simulink model "FullFMS_2026_02_25_V0_4_29_R2025b"  (R2025b)
settings: Solver=FixedStepAuto  StartTime=0.0  StopTime=inf  FixedStep=0.01  MaxStep=0.01  RelTol=1e-2
PreLoadFcn:
  | load("BUS_CONFIG.mat")
libraries: opcualib x8
(part 4 of 4)

== matlab function FullFMS_2026_02_25_V0_4_29_R2025b/MATLAB Function ==
  data: u1 input boolean; u2 input boolean; u3 input boolean; u4 input boolean; u5 input boolean; u6 input boolean; u7 input boolean; u8 input boolean; u9 input boolean; u10 input boolean; u11 input boolean; u12 input boolean; u13 input boolean; u14 input boolean; u15 input boolean; u16 input boolean; u17 input boolean; u18 input boolean; u19 input boolean; u20 input boolean; u21 input boolean; u22 input boolean; u23 input boolean; u24 input boolean; u25 input boolean; u26 input boolean; u27 input boolean; u28 input boolean; u29 input boolean; u30 input boolean; u31 input boolean; u32 input boolean; u33 input boolean; u34 input boolean; u35 input boolean; u36 input boolean; u37 input boolean; u38 input boolean; u39 input boolean; u40 input boolean; u41 input boolean; u42 input boolean; u43 input boolean; u44 input boolean; u45 input boolean; u46 input boolean; u47 input boolean; u48 input boolean; u49 input boolean; u50 input boolean; u51 input boolean; u52 input boolean; u53 input boolean; u54 input boolean; u55 input boolean; u56 input boolean; u57 input boolean; u58 input boolean; u59 input boolean; u60 input boolean; u61 input boolean; u62 input boolean; u63 input boolean; u64 input boolean; u65 input boolean; u66 input boolean; F_22_Led_On output boolean; F_22_Led_Off output boolean; F_22_Conveyor output boolean; F_24_Release_FB output boolean; F_25_Release_FB output boolean; F_26_Release_FB output boolean; F_27_Release_FB output boolean; F_28_Release_FB output boolean; F_29_Release_FB output boolean; C_24_CartDel output boolean; C_24_CRoute_Out output boolean; C_24_Request output boolean; C_24_CRoute_In output boolean; C_25_CartDel output boolean; C_25_CRoute_Out output boolean; C_25_Request output boolean; C_25_CRoute_In output boolean; C_26_CartDel output boolean; C_26_CRoute_Out output boolean; C_26_Request output boolean; C_26_CRoute_In output boolean; C_27_CartDel output boolean; C_27_CRoute_Out output boolean; C_27_Request output boolean; C_27_CRoute_In output boolean; C_28_CartDel output boolean; C_28_CRoute_Out output boolean; C_28_Request output boolean; C_28_CRoute_In output boolean; C_29_CartDel output boolean; C_29_CRoute_Out output boolean; C_29_Request output boolean; C_29_CRoute_In output boolean; O_20_On output boolean; O_20_Off output boolean; O_20_Controler_On output boolean; O_24_Cart_Stat output boolean; O_24_Cart_Next output boolean; O_24_Optic output boolean; O_24_Count output boolean; O_24_Pist_Bck output boolean; O_25_Cart_Stat output boolean; O_25_Cart_Next output boolean; O_25_Optic output boolean; O_25_Count output boolean; O_25_Pist_Bck output boolean; O_26_Cart_Stat output boolean; O_26_Cart_Next output boolean; O_26_Optic output boolean; O_26_Count output boolean; O_26_Pist_Bck output boolean; O_27_Cart_Stat output boolean; O_27_Cart_Next output boolean; O_27_Optic output boolean; O_27_Count output boolean; O_27_Pist_Bck output boolean; O_28_Cart_Stat output boolean; O_28_Cart_Next output boolean; O_28_Optic output boolean; O_28_Count output boolean; O_28_Pist_Bck output boolean; O_29_Cart_Stat output boolean; O_29_Cart_Next output boolean; O_29_Optic output boolean; O_29_Count output boolean; O_29_Pist_Bck output boolean
function [F_22_Led_On,F_22_Led_Off,F_22_Conveyor,F_24_Release_FB,F_25_Release_FB,F_26_Release_FB,F_27_Release_FB,F_28_Release_FB,F_29_Release_FB,...
 C_24_CartDel,C_24_CRoute_Out,C_24_Request,C_24_CRoute_In,C_25_CartDel,C_25_CRoute_Out,C_25_Request,C_25_CRoute_In,C_26_CartDel,C_26_CRoute_Out,C_26_Request,C_26_CRoute_In,C_27_CartDel,C_27_CRoute_Out,C_27_Request,C_27_CRoute_In,C_28_CartDel,C_28_CRoute_Out,C_28_Request,C_28_CRoute_In,C_29_CartDel,C_29_CRoute_Out,C_29_Request,C_29_CRoute_In,...
 O_20_On,O_20_Off,O_20_Controler_On,O_24_Cart_Stat,O_24_Cart_Next,O_24_Optic,O_24_Count,O_24_Pist_Bck,O_25_Cart_Stat,O_25_Cart_Next,O_25_Optic,O_25_Count,O_25_Pist_Bck,O_26_Cart_Stat,O_26_Cart_Next,O_26_Optic,O_26_Count,O_26_Pist_Bck,O_27_Cart_Stat,O_27_Cart_Next,O_27_Optic,O_27_Count,O_27_Pist_Bck,O_28_Cart_Stat,O_28_Cart_Next,O_28_Optic,O_28_Count,O_28_Pist_Bck,O_29_Cart_Stat,O_29_Cart_Next,O_29_Optic,O_29_Count,O_29_Pist_Bck] = ...
 MASTER_20 (u1, u2, u3, u4, u5, u6, u7, u8, u9, u10, u11, u12, u13, u14, u15, u16, u17, u18, u19, u20, u21, u22, u23, u24, u25, u26, u27, u28, u29, u30, u31, u32, u33, u34, u35, u36, u37, u38, u39, u40, u41, u42, u43, u44, u45, u46, u47, u48, u49, u50, u51, u52, u53, u54, u55, u56, u57, u58, u59, u60, u61, u62, u63, u64, u65, u66)

% Actuators (9 variables, starts at u1)
F_22_Led_On = u1;
F_22_Led_Off = u2;
F_22_Conveyor = u3;
F_24_Release_FB = u4;
F_25_Release_FB = u5;
F_26_Release_FB = u6;
F_27_Release_FB = u7;
F_28_Release_FB = u8;
F_29_Release_FB = u9;	

% Control (24 varaibles, starts at u10)
C_24_CartDel = u10;
C_24_CRoute_Out = u11;
C_24_Request = u12;
C_24_CRoute_In  = u13;
C_25_CartDel = u14;
C_25_CRoute_Out = u15;
C_25_Request = u16;
C_25_CRoute_In = u17;
C_26_CartDel = u18;
C_26_CRoute_Out = u19;
C_26_Request = u20;
C_26_CRoute_In = u21;
C_27_CartDel = u22;
C_27_CRoute_Out = u23;
C_27_Request = u24;
C_27_CRoute_In = u25;
C_28_CartDel = u26;
C_28_CRoute_Out = u27;
C_28_Request = u28;
C_28_CRoute_In = u29;
C_29_CartDel = u30;
C_29_CRoute_Out = u31;
C_29_Request = u32;
C_29_CRoute_In = u33;

% Sensors (33 variables, starts at u34)
O_20_On = u34;
O_20_Off = u35;
O_20_Controler_On = u36;
O_24_Cart_Stat = u37;
O_24_Cart_Next = u38;
O_24_Optic = u39;
O_24_Count = u40;
O_24_Pist_Bck = u41;
O_25_Cart_Stat = u42;
O_25_Cart_Next = u43;
O_25_Optic = u44;
O_25_Count = u45;
O_25_Pist_Bck = u46;
O_26_Cart_Stat = u47;
O_26_Cart_Next = u48;
O_26_Optic = u49;
O_26_Count = u50;
O_26_Pist_Bck = u51;
O_27_Cart_Stat = u52;
O_27_Cart_Next = u53;
O_27_Optic = u54;
O_27_Count = u55;
O_27_Pist_Bck = u56;
O_28_Cart_Stat = u57;
O_28_Cart_Next = u58;
O_28_Optic = u59;
O_28_Count = u60;
O_28_Pist_Bck = u61;
O_29_Cart_Stat = u62;
O_29_Cart_Next = u63;
O_29_Optic = u64;
O_29_Count = u65;
O_29_Pist_Bck = u66;

end

== matlab function FullFMS_2026_02_25_V0_4_29_R2025b/MATLAB Function1 ==
  data: u1 input boolean; u2 input boolean; u3 input boolean; u4 input boolean; u5 input boolean; u6 input boolean; u7 input boolean; u8 input boolean; u9 input boolean; u10 input boolean; u11 input double; u12 input boolean; u13 input boolean; u14 input boolean; u15 input boolean; u16 input boolean; u17 input boolean; u18 input boolean; u19 input boolean; u20 input boolean; u21 input boolean; u22 input boolean; u23 input boolean; u24 input boolean; u25 input boolean; u26 input boolean; u27 input boolean; u28 input boolean; u29 input boolean; u30 input boolean; u31 input boolean; u32 input boolean; u33 input boolean; F_33_Led_Start output boolean; F_33_Led_Reset output boolean; F_33_Led_Extra1 output boolean; F_33_Led_Extra2 output boolean; F_33_Spring_Cyl output boolean; F_33_Cover_Cyl output boolean; A_34_Request output boolean; A_34_No_Cart output boolean; A_34_Cart_Full output boolean; A_34_CRoute_Out output boolean; A_32_RoboCartID output double; A_34_Cart_Stat output boolean; A_34_Cart_Next output boolean; A_34_Optic output boolean; A_34_Count output boolean; A_34_Pist_Bck output boolean; A_34_Release_FB output boolean; A_34_CRoute_In output boolean; C_30_Robot1 output boolean; C_30_Robot2 output boolean; C_35_Part_Del output boolean; O_31_Start output boolean; O_31_Stop output boolean; O_31_Reset output boolean; O_31_Part_in_Claw output boolean; O_31_Orientation output boolean; O_32_Sp_Cyl_Bck output boolean; O_32_Sp_Cyl_Fwd output boolean; O_32_Co_Cyl_Bck output boolean; O_32_Co_Cyl_Fwd output boolean; O_32_Sp_PickUp output boolean; O_32_Co_PickUp output boolean; O_32_CoMag_Empty output boolean
function [F_33_Led_Start,F_33_Led_Reset,F_33_Led_Extra1,F_33_Led_Extra2,F_33_Spring_Cyl,F_33_Cover_Cyl,...
    A_34_Request,A_34_No_Cart,A_34_Cart_Full,A_34_CRoute_Out,A_32_RoboCartID,A_34_Cart_Stat,A_34_Cart_Next,A_34_Optic,A_34_Count,A_34_Pist_Bck,A_34_Release_FB,A_34_CRoute_In,...
    C_30_Robot1,C_30_Robot2,C_35_Part_Del,...
    O_31_Start,O_31_Stop,O_31_Reset,O_31_Part_in_Claw,O_31_Orientation,O_32_Sp_Cyl_Bck,O_32_Sp_Cyl_Fwd,O_32_Co_Cyl_Bck,O_32_Co_Cyl_Fwd,O_32_Sp_PickUp,O_32_Co_PickUp,O_32_CoMag_Empty] = ...
    Robot_30 (u1, u2, u3, u4, u5, u6, u7, u8, u9, u10, u11, u12, ...
    u13, u14, u15, u16, u17, u18, u19, u20, u21, u22, u23, u24, u25, u26, ...
    u27, u28, u29, u30, u31, u32, u33)

% Actuators (6 variables: starts at u1)
F_33_Led_Start = u1;
F_33_Led_Reset = u2;
F_33_Led_Extra1 = u3;
F_33_Led_Extra2 = u4;
F_33_Spring_Cyl = u5;
F_33_Cover_Cyl = u6;

% AS-i (12 variables: starts at u7)
A_34_Request = u7;
A_34_No_Cart = u8;
A_34_Cart_Full = u9;
A_34_CRoute_Out = u10;
A_32_RoboCartID = u11;
A_34_Cart_Stat = u12;
A_34_Cart_Next = u13;
A_34_Optic = u14;
A_34_Count = u15;
A_34_Pist_Bck = u16;
A_34_Release_FB = u17;
A_34_CRoute_In = u18;

% Control (3 variables: starts at u19)
C_30_Robot1 = u19;
C_30_Robot2 = u20;
C_35_Part_Del = u21;

% Sensors (12 variables: starts at u22)
O_31_Start = u22;
O_31_Stop = u23;
O_31_Reset = u24;
O_31_Part_in_Claw = u25;
O_31_Orientation = u26;
O_32_Sp_Cyl_Bck = u27;
O_32_Sp_Cyl_Fwd = u28;
O_32_Co_Cyl_Bck = u29;
O_32_Co_Cyl_Fwd = u30;
O_32_Sp_PickUp = u31;
O_32_Co_PickUp = u32;
O_32_CoMag_Empty = u33;

end

== matlab function FullFMS_2026_02_25_V0_4_29_R2025b/MATLAB Function2 ==
  data: u1 input boolean; u2 input boolean; u3 input boolean; u4 input boolean; u5 input boolean; u6 input boolean; u7 input boolean; u8 input boolean; u9 input boolean; u10 input boolean; u11 input boolean; u12 input boolean; u13 input boolean; u14 input boolean; u15 input boolean; u16 input boolean; u17 input double; u18 input boolean; u19 input boolean; u20 input boolean; u21 input boolean; u22 input boolean; u23 input boolean; u24 input boolean; u25 input boolean; u26 input boolean; u27 input boolean; u28 input boolean; u29 input boolean; u30 input boolean; u31 input boolean; u32 input boolean; u33 input boolean; u34 input boolean; u35 input boolean; u36 input boolean; u37 input boolean; u38 input boolean; u39 input boolean; u40 input boolean; u41 input boolean; u42 input boolean; u43 input boolean; u44 input boolean; F_52_Claw_2_Del output boolean; F_52_Claw_2_Cart output boolean; F_52_Claw_Down output boolean; F_52_Close_Claw output boolean; F_53_Led_Start output boolean; F_53_Led_Reset output boolean; F_53_Led_Extra1 output boolean; F_53_Led_Extra2 output boolean; F_53_Panel_O4 output boolean; F_53_Panel_O5 output boolean; F_53_Panel_O6 output boolean; F_53_Panel_O7 output boolean; A_54_Request output boolean; A_54_No_Cart output boolean; A_54_Cart_Full output boolean; A_54_CRoute_Out output boolean; A_53_SortCartID output double; A_54_Cart_Stat output boolean; A_54_Cart_Next output boolean; A_54_Optic output boolean; A_54_Count output boolean; A_54_Pist_Bck output boolean; A_54_Release_FB output boolean; A_54_CRoute_In output boolean; C_55_Initialization output boolean; C_55_PD_Sort output boolean; C_52_Profibus output boolean; C_55_Start output boolean; C_55_Cart2Del output boolean; O_50_Part_Reserve output boolean; O_50_Claw_Cart output boolean; O_50_Claw_Del output boolean; O_50_Claw_Reserve output boolean; O_50_Claw_Low output boolean; O_50_Claw_High output boolean; O_50_Part_in_Claw output boolean; O_51_Start output boolean; O_51_Stop output boolean; O_51_Key_Pos output boolean; O_51_Reset output boolean; O_51_Panel_I4 output boolean; O_51_Panel_I5 output boolean; O_51_Panel_I6 output boolean; O_51_Panel_I7 output boolean
function [F_52_Claw_2_Del, F_52_Claw_2_Cart,F_52_Claw_Down,F_52_Close_Claw,F_53_Led_Start,F_53_Led_Reset,F_53_Led_Extra1,F_53_Led_Extra2,F_53_Panel_O4,F_53_Panel_O5,F_53_Panel_O6,F_53_Panel_O7, ...
    A_54_Request,A_54_No_Cart,A_54_Cart_Full,A_54_CRoute_Out,A_53_SortCartID,A_54_Cart_Stat,A_54_Cart_Next,A_54_Optic,A_54_Count,A_54_Pist_Bck,A_54_Release_FB,A_54_CRoute_In, ...
    C_55_Initialization , C_55_PD_Sort , C_52_Profibus , C_55_Start , C_55_Cart2Del, ...
    O_50_Part_Reserve,O_50_Claw_Cart,O_50_Claw_Del,O_50_Claw_Reserve,O_50_Claw_Low,O_50_Claw_High,O_50_Part_in_Claw,O_51_Start,O_51_Stop,O_51_Key_Pos,O_51_Reset,O_51_Panel_I4,O_51_Panel_I5 , O_51_Panel_I6 , O_51_Panel_I7 ] = ...
    Handling1_50(u1, u2, u3, u4, u5, u6, u7, u8, u9, u10, u11, u12, ...
    u13, u14, u15, u16, u17, u18, u19, u20, u21, u22, u23, u24, u25, u26, ...
    u27, u28, u29, u30, u31, u32, u33, u34, u35, u36, u37, u38, u39, u40, ...
    u41, u42, u43, u44)

% Actuators (12 variables, starts at u1)
F_52_Claw_2_Del = u1;
F_52_Claw_2_Cart = u2;
F_52_Claw_Down = u3;
F_52_Close_Claw = u4;
F_53_Led_Start = u5;
F_53_Led_Reset = u6;
F_53_Led_Extra1 = u7;
F_53_Led_Extra2 = u8;
F_53_Panel_O4 = u9;
F_53_Panel_O5 = u10;
F_53_Panel_O6 = u11;
F_53_Panel_O7 = u12;

% AS-i (12 variables, starts at u13)
A_54_Request = u13;
A_54_No_Cart = u14;
A_54_Cart_Full = u15;
A_54_CRoute_Out = u16;
A_53_SortCartID = u17;
A_54_Cart_Stat = u18;
A_54_Cart_Next = u19;
A_54_Optic = u20;
A_54_Count = u21;
A_54_Pist_Bck = u22;
A_54_Release_FB = u23;
A_54_CRoute_In = u24;

% Control (5 variables, starts at u25)
C_55_Initialization = u25;
C_55_PD_Sort = u26;
C_52_Profibus = u27;
C_55_Start = u28;
C_55_Cart2Del = u29;

% Quarto bloco - Sensors (15 varaibles, starts at u30)
O_50_Part_Reserve = u30;
O_50_Claw_Cart = u31;
O_50_Claw_Del = u32;
O_50_Claw_Reserve = u33;
O_50_Claw_Low = u34;
O_50_Claw_High = u35;
O_50_Part_in_Claw = u36;
O_51_Start = u37;
O_51_Stop = u38;
O_51_Key_Pos = u39;
O_51_Reset = u40;
O_51_Panel_I4 = u41;
O_51_Panel_I5 = u42;
O_51_Panel_I6 = u43;
O_51_Panel_I7 = u44;

end

== matlab function FullFMS_2026_02_25_V0_4_29_R2025b/MATLAB Function3 ==
  data: F_62_Conveyor output boolean; F_62_P1 output boolean; F_62_P2 output boolean; F_62_Identify output boolean; F_63_Led_Start output boolean; F_63_Led_Reset output boolean; F_63_Led_Extra1 output boolean; F_63_Led_Extra2 output boolean; F_63_Panel_O4 output boolean; F_63_Panel_O5 output boolean; F_63_Panel_O6 output boolean; F_63_Panel_O7 output boolean; C_65_Initialization output boolean; C_65_ID_1 output boolean; C_65_ID_2 output boolean; C_65_Part_Sorted output boolean; C_62_Profibus output boolean; C_65_RBS_Output output boolean; C_65_RSB_Output output boolean; C_65_BRS_Output output boolean; C_65_BSR_Output output boolean; C_65_SRB_Output output boolean; C_65_SBR_Output output boolean; O_60_SPart output boolean; O_60_SInd output boolean; O_60_SPhoto output boolean; O_60_Part_Pass output boolean; O_60_SL1_Bck output boolean; O_60_SL1_Fwd output boolean; O_60_SL2_Bck output boolean; O_60_SL2_Fwd output boolean; O_61_Start output boolean; O_61_Stop output boolean; O_61_Key_Pos output boolean; O_61_Reset output boolean; O_61_Panel_I4 output boolean; O_61_Panel_I5 output boolean; O_61_Panel_I6 output boolean; O_61_Panel_I7 output boolean; u1 input boolean; u2 input boolean; u3 input boolean; u4 input boolean; u5 input boolean; u6 input boolean; u7 input boolean; u8 input boolean; u9 input boolean; u10 input boolean; u11 input boolean; u12 input boolean; u13 input boolean; u14 input boolean; u15 input boolean; u16 input boolean; u17 input boolean; u18 input boolean; u19 input boolean; u20 input boolean; u21 input boolean; u22 input boolean; u23 input boolean; u24 input boolean; u25 input boolean; u26 input boolean; u27 input boolean; u28 input boolean; u29 input boolean; u30 input boolean; u31 input boolean; u32 input boolean; u33 input boolean; u34 input boolean; u35 input boolean; u36 input boolean; u37 input boolean; u38 input boolean; u39 input boolean
function [F_62_Conveyor,F_62_P1,F_62_P2,F_62_Identify,F_63_Led_Start,F_63_Led_Reset,F_63_Led_Extra1,F_63_Led_Extra2,F_63_Panel_O4,F_63_Panel_O5,F_63_Panel_O6,F_63_Panel_O7, ...
C_65_Initialization,C_65_ID_1,C_65_ID_2,C_65_Part_Sorted,C_62_Profibus,C_65_RBS_Output,C_65_RSB_Output,C_65_BRS_Output,C_65_BSR_Output,C_65_SRB_Output,C_65_SBR_Output, ...
O_60_SPart,O_60_SInd,O_60_SPhoto,O_60_Part_Pass,O_60_SL1_Bck,O_60_SL1_Fwd,O_60_SL2_Bck,O_60_SL2_Fwd,O_61_Start,O_61_Stop,O_61_Key_Pos,O_61_Reset,O_61_Panel_I4,O_61_Panel_I5,O_61_Panel_I6,O_61_Panel_I7] = ...
Sorintg_60 (u1, u2, u3, u4, u5, u6, u7, u8, u9, u10, u11, u12, u13, u14, u15, u16, u17, u18, u19, u20, u21, u22, u23, u24, u25, u26, u27, u28, u29, u30, u31, u32, u33, u34, u35, u36, u37, u38, u39)

% Actuators (12 variables, starts at u1)
F_62_Conveyor = u1;
F_62_P1 = u2;
F_62_P2 = u3;
F_62_Identify = u4;
F_63_Led_Start = u5;
F_63_Led_Reset = u6;
F_63_Led_Extra1 = u7;
F_63_Led_Extra2 = u8;
F_63_Panel_O4 = u9;
F_63_Panel_O5 = u10;
F_63_Panel_O6 = u11;
F_63_Panel_O7 = u12;

% Control (11 variables, starts at u13)
C_65_Initialization = u13;
C_65_ID_1 = u14;
C_65_ID_2 = u15;
C_65_Part_Sorted = u16;
C_62_Profibus = u17;
C_65_RBS_Output = u18;
C_65_RSB_Output = u19;
C_65_BRS_Output = u20;
C_65_BSR_Output = u21;
C_65_SRB_Output = u22;
C_65_SBR_Output = u23;

% Sensors (16 varaibles, starts at u24)
O_60_SPart = u24;
O_60_SInd = u25;
O_60_SPhoto = u26;
O_60_Part_Pass = u27;
O_60_SL1_Bck = u28;
O_60_SL1_Fwd = u29;
O_60_SL2_Bck = u30;
O_60_SL2_Fwd = u31;
O_61_Start = u32;
O_61_Stop = u33;
O_61_Key_Pos = u34;
O_61_Reset = u35;
O_61_Panel_I4 = u36;
O_61_Panel_I5 = u37;
O_61_Panel_I6 = u38;
O_61_Panel_I7 = u39;

end
